simulink model "ts_b02f_log"  (R2024b)
settings: Solver=FixedStepDiscrete  StartTime=0.0  StopTime=10  FixedStep=Ts  RelTol=1e-4
PreLoadFcn:
  | Ts=50e-6;
undefined symbols (not defined in the file): D1, Delta, DiscIntNeverNeededParam
libraries: simulink x22, spsSecondOrderFilterLib x14, spsThreePhaseVIMeasurementLib x7, spsabctodq0Lib x6, spsThreePhaseSeriesRLCLoadLib x5, spsPowerPLLDrivenPositiveSequenceLib x4, spsStairGeneratorLib x4, spsThreePhaseTransformerTwoWindingsLib x3, spsDCVoltageSourceLib x3, spsThreePhaseSeriesRLCBranchLib x3, spsPWMGeneratorPulseAveragingLib x3, spsTwoLevelConverterLib x3
(part 1 of 3)
settings Model: Creator=The MathWorks, Inc.  LastModifiedBy=sande
settings SolverCC: AlgebraicLoopSolver=TrustRegion
settings DataIOCC: SaveOutput=off  DSMLogging=off  SaveTime=off  ReturnWorkspaceOutputs=off  SignalLoggingName=SignalLog
settings DebuggingCC: UnconnectedInputMsg=warning  UnconnectedOutputMsg=warning  UnconnectedLineMsg=warning  ArithmeticOperatorsInVariantConditions=warning
settings ModelReferenceCC: EnableRefExpFcnMdlSchedulingChecks=on
settings SFSimCC: CustomCodeUndefinedFunction=UseInterfaceOnly
settings RTWCC: GPUComputeCapability=3.5  DLArmComputeVersion=19.05

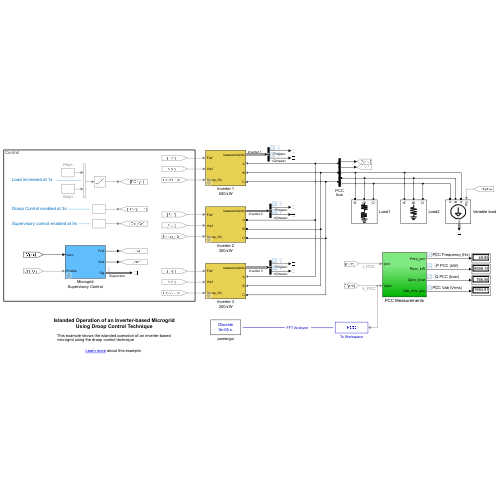
[thumbnail: Simulink's stored preview of the top-level diagram]
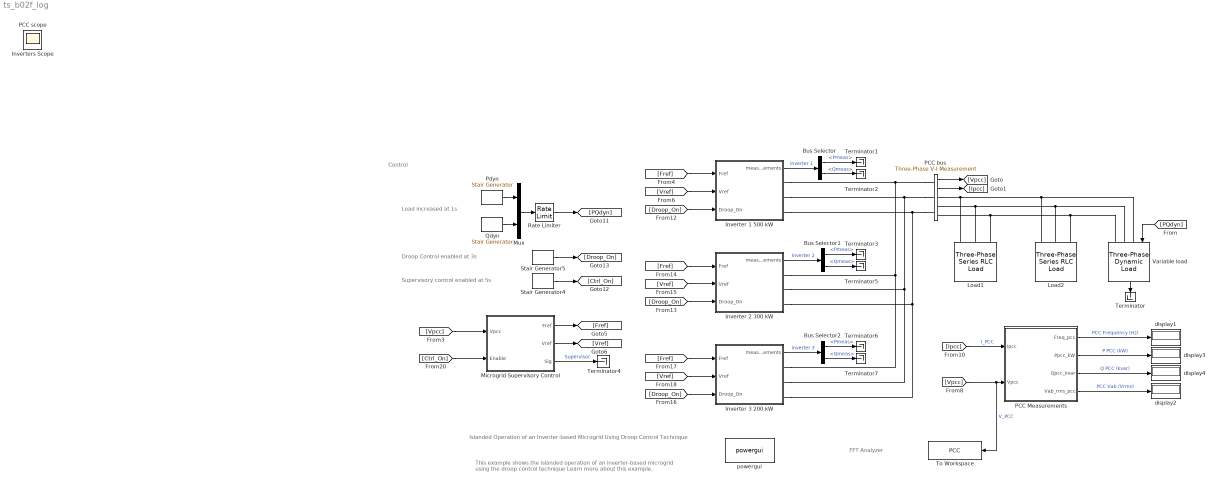
== system ts_b02f_log ==
  note: This example shows the islanded operation of an inverter-based microgrid using the droop control technique
      |
      | Learn more about this example.
  note: FFT Analyzer
  note: Control
  note: Islanded Operation of an Inverter-based Microgrid
      | Using Droop Control Technique
  note: Load increased at 1s
  note: Supervisory control enabled at 5s
  note: Droop Control enabled at 3s
  Bus Selector : BusSelector  OutputSignals=Control.Pmeas,Control.Qmeas
  Bus Selector1 : BusSelector  OutputSignals=Control.Pmeas,Control.Qmeas
  Bus Selector2 : BusSelector  OutputSignals=Control.Pmeas,Control.Qmeas
  Inverter 1 500 kW : Subsystem  mask(Grid-Forming Inverter with droop control){Pnom=5.874e+06, Fnom=50, Vnom_prim=22e3, Vnom_sec=480, Vnom_dc=1000, Frequency_Droop=1, Voltage_Droop=4, Kp_Vreg=2, Ki_Vreg=14, Kp_Ireg=0.3, Ki_Ireg=20, RLff=[ 0.004, 0.21], Fsw=2700, CarrierPhase=90, fn_Filter=500, Ts=Ts}
      mask prompts: Pnom "Power (VA)"; Fnom "Frequency (Hz)"; Vnom_prim "Primary line voltage (Vrms)"; Vnom_sec "Secondary line voltage (Vrms)"; Vnom_dc "DC link voltage (V)"; Frequency_Droop "Frequency droop (%)"; Voltage_Droop "Voltage droop (%)"; Kp_Vreg "Proportional gain"; Ki_Vreg "Integral gain"; Kp_Ireg "Proportional gain"; Ki_Ireg "Integral gain"; RLff "Feedforward coefficients (pu)"; Fsw "Switching frequency (Hz)"; CarrierPhase "Carrier initial phase (degrees)"; fn_Filter "Measurement filters fn (Hz)"; Ts "Sample time (s)"
      mask init:
      | Rff=RLff(1);
      | Lff=RLff(2);
      mask DialogControl Container4 Prompt: Nominal Values:
      mask DialogControl Container8 Prompt: Droop Values
      mask DialogControl Container7 Prompt: Voltage Regulators
      mask DialogControl Container10 Prompt: Current Regulators
      mask DialogControl Ts1 Prompt: PWM Generator
  Inverter 2 300 kW : Subsystem  mask(Grid-Forming Inverter with droop control){Pnom=5.874e+06, Fnom=50, Vnom_prim=22e3, Vnom_sec=480, Vnom_dc=1000, Frequency_Droop=1, Voltage_Droop=4, Kp_Vreg=2, Ki_Vreg=10, Kp_Ireg=0.3, Ki_Ireg=20, RLff=[ 0.004, 0.21], Fsw=2700, CarrierPhase=90, fn_Filter=500, Ts=Ts}
      mask prompts: Pnom "Power (VA)"; Fnom "Frequency (Hz)"; Vnom_prim "Primary line voltage (Vrms)"; Vnom_sec "Secondary line voltage (Vrms)"; Vnom_dc "DC link voltage (V)"; Frequency_Droop "Frequency droop (%)"; Voltage_Droop "Voltage droop (%)"; Kp_Vreg "Proportional gain"; Ki_Vreg "Integral gain"; Kp_Ireg "Proportional gain"; Ki_Ireg "Integral gain"; RLff "Feedforward coefficients (pu)"; Fsw "Switching frequency (Hz)"; CarrierPhase "Carrier initial phase (degrees)"; fn_Filter "Measurement filters fn (Hz)"; Ts "Sample time (s)"
      mask init:
      | Rff=RLff(1);
      | Lff=RLff(2);
      mask DialogControl Container4 Prompt: Nominal Values:
      mask DialogControl Container8 Prompt: Droop Values
      mask DialogControl Container7 Prompt: Voltage Regulators
      mask DialogControl Container10 Prompt: Current Regulators
      mask DialogControl Ts1 Prompt: PWM Generator
  Inverter 3 200 kW : Subsystem  mask(Grid-Forming Inverter with droop control){Pnom=5.874e+06, Fnom=50, Vnom_prim=22e3, Vnom_sec=480, Vnom_dc=1000, Frequency_Droop=1, Voltage_Droop=4, Kp_Vreg=2, Ki_Vreg=12, Kp_Ireg=0.3, Ki_Ireg=20, RLff=[ 0.004, 0.21], Fsw=2340, CarrierPhase=0, fn_Filter=500, Ts=Ts}
      mask prompts: Pnom "Power (VA)"; Fnom "Frequency (Hz)"; Vnom_prim "Primary line voltage (Vrms)"; Vnom_sec "Secondary line voltage (Vrms)"; Vnom_dc "DC link voltage (V)"; Frequency_Droop "Frequency droop (%)"; Voltage_Droop "Voltage droop (%)"; Kp_Vreg "Proportional gain"; Ki_Vreg "Integral gain"; Kp_Ireg "Proportional gain"; Ki_Ireg "Integral gain"; RLff "Feedforward coefficients (pu)"; Fsw "Switching frequency (Hz)"; CarrierPhase "Carrier initial phase (degrees)"; fn_Filter "Measurement filters fn (Hz)"; Ts "Sample time (s)"
      mask init:
      | Rff=RLff(1);
      | Lff=RLff(2);
      mask DialogControl Container4 Prompt: Nominal Values:
      mask DialogControl Container8 Prompt: Droop Values
      mask DialogControl Container7 Prompt: Voltage Regulators
      mask DialogControl Container10 Prompt: Current Regulators
      mask DialogControl Ts1 Prompt: PWM Generator
  Load1 : spsThreePhaseSeriesRLCLoadLib/Three-Phase Series RLC Load  LConnTagsString=A|B|C  Configuration=Y (grounded)  NominalVoltage=22e3  Vabc=[1e3 1e3 1e3]  Vabcp=[1e3 1e3 1e3]  NominalFrequency=50  UnbalancedPower=off  ActivePower=5e6  InductivePower=388172  CapacitivePower=0  Pabc=[10e3 9e3 11e3]  QLabc=[100 90 110]  QCabc=[100 90 110]  Pabcp=[10e3 9e3 11e3]  QLabcp=[100 90 110]  QCabcp=[100 90 110]  Measurements=None  LoadType=constant Z
  Load2 : spsThreePhaseSeriesRLCLoadLib/Three-Phase Series RLC Load  LConnTagsString=A|B|C  Configuration=Y (grounded)  NominalVoltage=22e3  Vabc=[1e3 1e3 1e3]  Vabcp=[1e3 1e3 1e3]  NominalFrequency=50  UnbalancedPower=off  ActivePower=0.05e6  InductivePower=0  CapacitivePower=0  Pabc=[10e3 9e3 11e3]  QLabc=[100 90 110]  QCabc=[100 90 110]  Pabcp=[10e3 9e3 11e3]  QLabcp=[100 90 110]  QCabcp=[100 90 110]  Measurements=None  LoadType=constant Z
  Microgrid Supervisory Control : Subsystem  mask(Microgrid Supervisory Control){Fnom=50, Vnom=22e3, Kp_Freg=0.03, Ki_Freg=2, Freg_Limits=[1.02, 0.98] * 50, Kp_Vreg=0.1, Ki_Vreg=7, Vreg_Limits=[1.04, 0.96] * 22e3, fn_Filter=10, Ts=Ts}
      mask prompts: Fnom "Frequency (Hz)"; Vnom "Line voltage (Vrms)"; Kp_Freg "Proportional gain"; Ki_Freg "Integral gain"; Freg_Limits "Output limits (Hz): [Upper Lower]"; Kp_Vreg "Proportional gain"; Ki_Vreg "Integral gain"; Vreg_Limits "Output limits (Hz): [Upper Lower]"; fn_Filter "Measurement filter fn (Hz)"; Ts "Sample time (s)"
      mask DialogControl Container4 Prompt: Nominal Values:
      mask DialogControl Container7 Prompt: Frequency Regulator
      mask DialogControl Container10 Prompt: Voltage Regulator
  Mux : Mux  Inputs=2
  PCC bus : spsThreePhaseVIMeasurementLib/Three-Phase V-I Measurement  VoltageMeasurement=phase-to-ground  SetLabelV=off  LabelV=Vabc  Vpu=off  VpuLL=off  CurrentMeasurement=yes  SetLabelI=off  LabelI=Iabc  Ipu=off  Pbase=100e6  Vbase=500e3  OutputType=Complex  PhasorSimulation=off  PSBequivalent=0
  PCC Measurements : Subsystem
  Pdyn : spsStairGeneratorLib/Stair Generator  t=[0, 1]  e=[0 4.95e6]  Ts=Ts
  Qdyn : spsStairGeneratorLib/Stair Generator  t=[0, 1]  e=[0 388172]  Ts=Ts
  Rate Limiter : RateLimiter  RisingSlewLimit=6.2e6  FallingSlewLimit=-6.2e6  SampleTimeMode=inherited
  Stair Generator4 : spsStairGeneratorLib/Stair Generator  t=[0, 5]  e=[0, 1]  Ts=Ts
  Stair Generator5 : spsStairGeneratorLib/Stair Generator  t=[0, 3]  e=[0, 1]  Ts=Ts
  Terminator{,1..7} (8 alike) : Terminator
  To Workspace : ToWorkspace  VariableName=PCC  SaveFormat=Structure With Time  SampleTime=-1
  Variable load : spsThreePhaseDynamicLoadLib/Three-Phase Dynamic Load  NominalVoltage=[ 22e3 50 ]  ActiveReactivePowers=[1e6 0]  PositiveSequence=[1 0]  ExternalControl=on  NpNq=[1.3 2]  TimeConstants="[0  0  0  0]"  MinimumVoltage=0.7  Tfilter=1e-4  LoadFlowParameters=[4,0,0,0,0]
      link override Model/PLL/Second-Order Filter: Vac_Init=[0, 0, 50]
  display{1..4} (4 alike) : Display
      settings: Format=bank  Decimation=500
  powergui : spspowerguiLib/powergui  Priority=2  SimulationMode=Discrete  SampleTime=Ts  frequency=50  Iterations=50  frequencyindice=0  Pbase=100e6  ErrMax=1e-4  UnitsV=kV  UnitsW=MW  buscounter=0  FunctionMessages=off  echomessages=off  EnableUseOfTLC=off  CurrentSourceSwitches=off  DisableSnubberDevices=off  DisableRonSwitches=off  DisableVfSwitches=off  DisplayEquations=off  AutomaticDiscreteSolvers=off  SolverType=Tustin/Backward Euler (TBE)  Interpol=off  ExternalGateDelay=off  methode=off  Ts=0  x0status=blocks  SPID=off  SwTol=0  HookPort=off  NonlinearTolerance=1e-4  nMaxIteration=100  ContinueOnMaxIteration=on  RestoreLinks=warning  ResistiveCurrentMeasurement=off  Frange=[0:2:500]  Ylog=off  Xlog=off  ShowGrid=off  save=off  variable=ZData  structure=ScopeData_VIpcc  ZoomFFT=on  StartTime=6.8  cycles=1  DisplayStyle=1  fundamental=50  FreqAxis=off  MaxFrequency=7000  frequencyindicesteady=1  RmsSteady=1  display=off
  Inverters Scope : Scope
  PCC scope : Scope
  wires:
  [Vref] -> Inverter 1 500 kW/2(Vref)
  [Fref] -> Inverter 1 500 kW/1(Fref)
  PCC bus/1 -> [Vpcc]
  PCC bus/2 -> [Ipcc]
  [Vpcc] -> Microgrid Supervisory Control/1(Vpcc)
  Microgrid Supervisory Control/1(Fref) -> [Fref]
  Microgrid Supervisory Control/2(Vref) -> [Vref]
  Microgrid Supervisory Control/3(Sig) -> Terminator4/1  "Supervisor"
  [Ipcc] -> PCC Measurements/1(Ipcc)  "I_PCC"
  [Vpcc] -> To Workspace/1, PCC Measurements/2(Vpcc)  "V_PCC"
  PCC Measurements/1(Freq_pcc) -> display1/1  "PCC Frequency (Hz)"
  PCC Measurements/4(Vab_rms_pcc) -> display2/1  "PCC Vab (Vrms)"
  [Droop_On] -> Inverter 1 500 kW/3(Droop_On)
  [Fref] -> Inverter 2 300 kW/1(Fref)
  [Vref] -> Inverter 2 300 kW/2(Vref)
  [Droop_On] -> Inverter 2 300 kW/3(Droop_On)
  [Fref] -> Inverter 3 200 kW/1(Fref)
  [Vref] -> Inverter 3 200 kW/2(Vref)
  [Droop_On] -> Inverter 3 200 kW/3(Droop_On)
  [Ctrl_On] -> Microgrid Supervisory Control/2(Enable)
  Variable load/1 -> Terminator/1
  [PQdyn] -> Variable load/1
  Mux/1 -> Rate Limiter/1
  Pdyn/1 -> Mux/1
  Qdyn/1 -> Mux/2
  Stair Generator5/1 -> [Droop_On]
  Stair Generator4/1 -> [Ctrl_On]
  Rate Limiter/1 -> [PQdyn]
  Inverter 1 500 kW/1(measurements) -> Bus Selector/1  "inverter 1"
  Inverter 2 300 kW/1(measurements) -> Bus Selector1/1  "inverter 2"
  Inverter 3 200 kW/1(measurements) -> Bus Selector2/1  "inverter 3"
  PCC Measurements/2(Ppcc_kW) -> display3/1  "P PCC (kW)"
  PCC Measurements/3(Qpcc_kvar) -> display4/1  "Q PCC (kvar)"
  Bus Selector/1 -> Terminator1/1  "<Pmeas>"
  Bus Selector/2 -> Terminator2/1  "<Qmeas>"
  Bus Selector1/1 -> Terminator3/1  "<Pmeas>"
  Bus Selector1/2 -> Terminator5/1  "<Qmeas>"
  Bus Selector2/1 -> Terminator6/1  "<Pmeas>"
  Bus Selector2/2 -> Terminator7/1  "<Qmeas>"
  connections:
  Load1/LConn1 -- Load2/LConn1 -- Variable load/LConn1 -- PCC bus/RConn1
  Load1/LConn2 -- Load2/LConn2 -- Variable load/LConn2 -- PCC bus/RConn2
  Load1/LConn3 -- Load2/LConn3 -- Variable load/LConn3 -- PCC bus/RConn3
  PCC bus/LConn2 -- Inverter 1 500 kW/RConn2 -- Inverter 2 300 kW/RConn2 -- Inverter 3 200 kW/RConn2
  PCC bus/LConn3 -- Inverter 1 500 kW/RConn3 -- Inverter 2 300 kW/RConn3 -- Inverter 3 200 kW/RConn3
  PCC bus/LConn1 -- Inverter 1 500 kW/RConn1 -- Inverter 2 300 kW/RConn1 -- Inverter 3 200 kW/RConn1

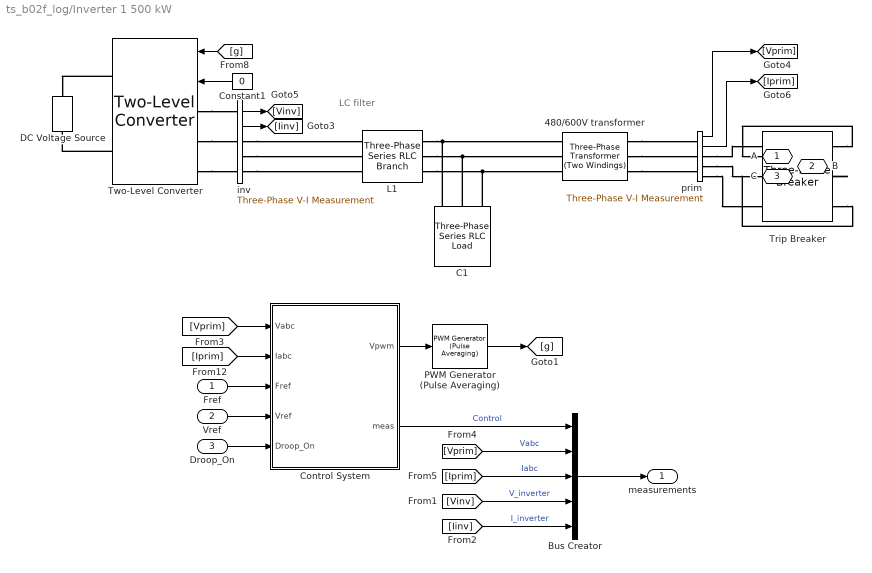
== system ts_b02f_log/Inverter 1 500 kW ==
  note: LC filter
  Fref : Inport  PortDimensions=1
  Vref : Inport  Port=2  PortDimensions=1
  Droop_On : Inport  Port=3  PortDimensions=1
  480/600V transformer : spsThreePhaseTransformerTwoWindingsLib/Three-Phase Transformer (Two Windings)  Winding1Connection=Yg  Winding2Connection=Delta (D1)  CoreType=Three single-phase transformers  SetSaturation=off  Hysteresis=off  DataFile='hysteresis'  SetInitialFlux=off  Measurements=None  UNITS=pu  NominalPower=[Pnom*1.1 , Fnom ]  Winding1=[ Vnom_prim , 0.0015 , 0.03]  Winding2=[Vnom_sec , 0.0015 , 0.03 ]  Rm=200  Lm=200  L0=0.5  Saturation=[ 0,0 ; 0.0024,1.2 ; 1.0,1.52 ]  InitialFluxes=[ 0.8 , -0.8 , 0.7 ]  BreakLoop=off  DiscreteSolver=Trapezoidal iterative  DataType=off  TransfoNumber=0
  Bus Creator : BusCreator  Inputs=5
  C1 : spsThreePhaseSeriesRLCLoadLib/Three-Phase Series RLC Load  LConnTagsString=A|B|C  Configuration=Y (grounded)  NominalVoltage=Vnom_sec  Vabc=[1e3 1e3 1e3]  Vabcp=[1e3 1e3 1e3]  NominalFrequency=Fnom  UnbalancedPower=off  ActivePower=0.05*Pnom/50  InductivePower=0  CapacitivePower=0.05*Pnom  Pabc=[10e3 9e3 11e3]  QLabc=[100 90 110]  QCabc=[100 90 110]  Pabcp=[10e3 9e3 11e3]  QLabcp=[100 90 110]  QCabcp=[100 90 110]  Measurements=None  LoadType=constant Z
  Constant1 : Constant  Value=0
  Control System : Subsystem  mask(Inverter Control){Pnom=Pnom, Fnom=Fnom, Vnom_prim=Vnom_prim, Vnom_sec=Vnom_sec, Vnom_dc=Vnom_dc, Frequency_Droop=Frequency_Droop, Voltage_Droop=Voltage_Droop, Kp_Vreg=Kp_Vreg, Ki_Vreg=Ki_Vreg, fn_Filter=fn_Filter, Kp_Ireg=Kp_Ireg, Ki_Ireg=Ki_Ireg, RLff=[ Rff Lff], Ts=Ts}
      mask prompts: Pnom "Power (VA)"; Fnom "Frequency (Hz)"; Vnom_prim "Primary voltage (Vrms)"; Vnom_sec "Secondary voltage (Vrms)"; Vnom_dc "DC voltage (V)"; Frequency_Droop "Frequency droop (%)"; Voltage_Droop "Voltage droop (%)"; Kp_Vreg "Proportional gain"; Ki_Vreg "Integral gain"; fn_Filter "Measurement filter fn (Hz)"; Kp_Ireg "Proportional gain"; Ki_Ireg "Integral gain"; RLff "Feedforward Values [Rff Lff] (pu)"; Ts "Control sample time:"
      mask init:
      | Rff=RLff(1);
      | Lff=RLff(2);
      | Limits_Ireg=[1.25, -1.25];
      | Limits_Vreg=[1.25, -1.25];
      mask DialogControl Container4 Prompt: Nominal Values:
      mask DialogControl Container8 Prompt: Droop Values
      mask DialogControl Container9 Prompt: Voltage regulators
      mask DialogControl Container6 Prompt: Current regulators:
      mask DialogControl Ts1 Prompt: Sample time (s)
  DC Voltage Source : spsDCVoltageSourceLib/DC Voltage Source  Amplitude=1000  Measurements=None
  L1 : spsThreePhaseSeriesRLCBranchLib/Three-Phase Series RLC Branch  LConnTagsString=A|B|C  RConnTagsString=A|B|C  BranchType=RL  Resistance=0.15 * (Vnom_sec^2/Pnom)/100  Inductance=0.15 * (Vnom_sec^2/Pnom/2/pi/Fnom)  Capacitance=inf  Measurements=None
  PWM Generator (Pulse Averaging) : spsPWMGeneratorPulseAveragingLib/PWM Generator (Pulse Averaging)  GeneratorType=Two-level, three-phase  Fc=Fsw  InitialPhase=CarrierPhase  Ts=Ts
  Trip Breaker : spsThreePhaseBreakerLib/Three-Phase Breaker  InitialState=closed  SwitchA=on  SwitchB=on  SwitchC=on  SwitchTimes=[6]  External=off  BreakerResistance=0.01  SnubberResistance=1e6  SnubberCapacitance=inf  Measurements=None
  Two-Level Converter : spsTwoLevelConverterLib/Two-Level Converter  ModelType=Switching function  Ron=1e-3  Rs=1e6  Cs=inf  Vforward=[0,0]  Ron_Diode=1e-3  Rs_Diode=1e6  Cs_Diode=inf  Vf_Diode=0  Rs_CurrentSource=inf  Ron_ACsource=1e-3
  inv : spsThreePhaseVIMeasurementLib/Three-Phase V-I Measurement  VoltageMeasurement=phase-to-ground  SetLabelV=off  LabelV=Vabc_B1  Vpu=off  VpuLL=off  CurrentMeasurement=yes  SetLabelI=off  LabelI=Iabc_B1  Ipu=off  Pbase=100e6  Vbase=500e3  OutputType=Magnitude  PhasorSimulation=off  PSBequivalent=0
  prim : spsThreePhaseVIMeasurementLib/Three-Phase V-I Measurement  VoltageMeasurement=phase-to-ground  SetLabelV=off  LabelV=Vabc_B1  Vpu=off  VpuLL=off  CurrentMeasurement=yes  SetLabelI=off  LabelI=Iabc_B1  Ipu=off  Pbase=100e6  Vbase=500e3  OutputType=Magnitude  PhasorSimulation=off  PSBequivalent=0
  A : PMIOPort  Side=Right
  B : PMIOPort  Port=2  Side=Right
  C : PMIOPort  Port=3  Side=Right
  measurements : Outport
  wires:
  Bus Creator/1 -> measurements/1
  [Iinv] -> Bus Creator/5  "I_inverter"
  [Vinv] -> Bus Creator/4  "V_inverter"
  [Iprim] -> Bus Creator/3  "Iabc"
  [Vprim] -> Bus Creator/2  "Vabc"
  Control System/1(Vpwm) -> PWM Generator (Pulse Averaging)/1
  inv/2 -> [Iinv]
  PWM Generator (Pulse Averaging)/1 -> [g]
  inv/1 -> [Vinv]
  [g] -> Two-Level Converter/1
  Constant1/1 -> Two-Level Converter/2
  Fref/1 -> Control System/3(Fref)
  Vref/1 -> Control System/4(Vref)
  Control System/2(meas) -> Bus Creator/1  "Control"
  Droop_On/1 -> Control System/5(Droop_On)
  prim/2 -> [Iprim]
  prim/1 -> [Vprim]
  [Vprim] -> Control System/1(Vabc)
  [Iprim] -> Control System/2(Iabc)
  connections:
  L1/RConn2 -- 480/600V transformer/RConn2 -- C1/LConn2
  L1/RConn1 -- 480/600V transformer/RConn1 -- C1/LConn1
  L1/RConn3 -- 480/600V transformer/RConn3 -- C1/LConn3
  Two-Level Converter/RConn1 -- DC Voltage Source/RConn1
  inv/RConn3 -- L1/LConn3
  Two-Level Converter/LConn3 -- inv/LConn3
  inv/RConn1 -- L1/LConn1
  Two-Level Converter/LConn2 -- inv/LConn2
  inv/RConn2 -- L1/LConn2
  Two-Level Converter/LConn1 -- inv/LConn1
  Two-Level Converter/RConn2 -- DC Voltage Source/LConn1
  480/600V transformer/LConn2 -- prim/LConn2
  480/600V transformer/LConn1 -- prim/LConn1
  480/600V transformer/LConn3 -- prim/LConn3
  prim/RConn1 -- Trip Breaker/LConn1
  Trip Breaker/RConn1 -- A/RConn1
  prim/RConn2 -- Trip Breaker/LConn2
  Trip Breaker/RConn2 -- B/RConn1
  prim/RConn3 -- Trip Breaker/LConn3
  Trip Breaker/RConn3 -- C/RConn1

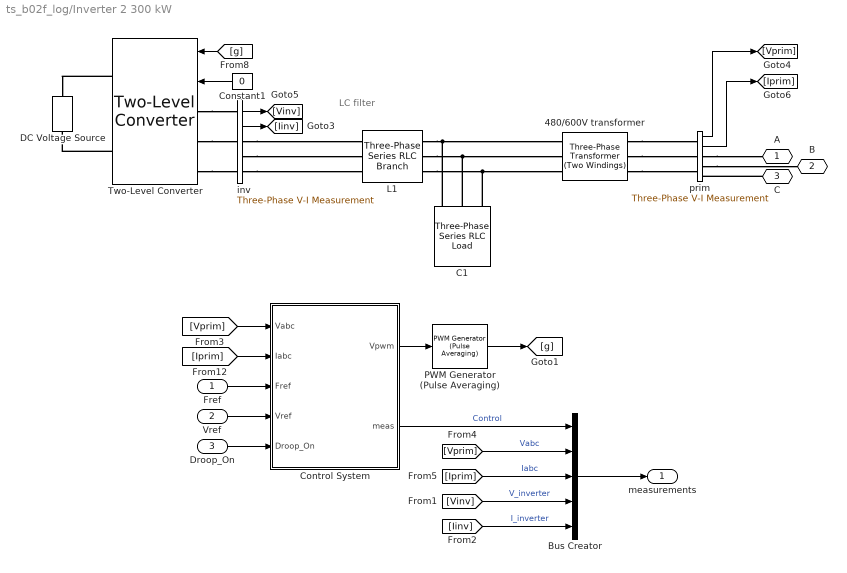
== system ts_b02f_log/Inverter 2 300 kW ==
  note: LC filter
  Fref : Inport  PortDimensions=1
  Vref : Inport  Port=2  PortDimensions=1
  Droop_On : Inport  Port=3  PortDimensions=1
  480/600V transformer : spsThreePhaseTransformerTwoWindingsLib/Three-Phase Transformer (Two Windings)  Winding1Connection=Yg  Winding2Connection=Delta (D1)  CoreType=Three single-phase transformers  SetSaturation=off  Hysteresis=off  DataFile='hysteresis'  SetInitialFlux=off  Measurements=None  UNITS=pu  NominalPower=[Pnom*1.1 , Fnom ]  Winding1=[ Vnom_prim , 0.0015 , 0.03]  Winding2=[Vnom_sec , 0.0015 , 0.03 ]  Rm=200  Lm=200  L0=0.5  Saturation=[ 0,0 ; 0.0024,1.2 ; 1.0,1.52 ]  InitialFluxes=[ 0.8 , -0.8 , 0.7 ]  BreakLoop=off  DiscreteSolver=Trapezoidal iterative  DataType=off  TransfoNumber=0
  Bus Creator : BusCreator  Inputs=5
  C1 : spsThreePhaseSeriesRLCLoadLib/Three-Phase Series RLC Load  LConnTagsString=A|B|C  Configuration=Y (grounded)  NominalVoltage=Vnom_sec  Vabc=[1e3 1e3 1e3]  Vabcp=[1e3 1e3 1e3]  NominalFrequency=Fnom  UnbalancedPower=off  ActivePower=0.05*Pnom/50  InductivePower=0  CapacitivePower=0.05*Pnom  Pabc=[10e3 9e3 11e3]  QLabc=[100 90 110]  QCabc=[100 90 110]  Pabcp=[10e3 9e3 11e3]  QLabcp=[100 90 110]  QCabcp=[100 90 110]  Measurements=None  LoadType=constant Z
  Constant1 : Constant  Value=0
  Control System : Subsystem  mask(Inverter Control){Pnom=Pnom, Fnom=Fnom, Vnom_prim=Vnom_prim, Vnom_sec=Vnom_sec, Vnom_dc=Vnom_dc, Frequency_Droop=Frequency_Droop, Voltage_Droop=Voltage_Droop, Kp_Vreg=Kp_Vreg, Ki_Vreg=Ki_Vreg, fn_Filter=fn_Filter, Kp_Ireg=Kp_Ireg, Ki_Ireg=Ki_Ireg, RLff=[ Rff Lff], Ts=Ts}
      mask prompts: Pnom "Power (VA)"; Fnom "Frequency (Hz)"; Vnom_prim "Primary voltage (Vrms)"; Vnom_sec "Secondary voltage (Vrms)"; Vnom_dc "DC voltage (V)"; Frequency_Droop "Frequency droop (%)"; Voltage_Droop "Voltage droop (%)"; Kp_Vreg "Proportional gain"; Ki_Vreg "Integral gain"; fn_Filter "Measurement filter fn (Hz)"; Kp_Ireg "Proportional gain"; Ki_Ireg "Integral gain"; RLff "Feedforward Values [Rff Lff] (pu)"; Ts "Control sample time:"
      mask init:
      | Rff=RLff(1);
      | Lff=RLff(2);
      | Limits_Ireg=[1.25, -1.25];
      | Limits_Vreg=[1.25, -1.25];
      mask DialogControl Container4 Prompt: Nominal Values:
      mask DialogControl Container8 Prompt: Droop Values
      mask DialogControl Container9 Prompt: Voltage regulators
      mask DialogControl Container6 Prompt: Current regulators:
      mask DialogControl Ts1 Prompt: Sample time (s)
  DC Voltage Source : spsDCVoltageSourceLib/DC Voltage Source  Amplitude=1000  Measurements=None
  L1 : spsThreePhaseSeriesRLCBranchLib/Three-Phase Series RLC Branch  LConnTagsString=A|B|C  RConnTagsString=A|B|C  BranchType=RL  Resistance=0.15 * (Vnom_sec^2/Pnom)/100  Inductance=0.15 * (Vnom_sec^2/Pnom/2/pi/Fnom)  Capacitance=inf  Measurements=None
  PWM Generator (Pulse Averaging) : spsPWMGeneratorPulseAveragingLib/PWM Generator (Pulse Averaging)  GeneratorType=Two-level, three-phase  Fc=Fsw  InitialPhase=CarrierPhase  Ts=Ts
  Two-Level Converter : spsTwoLevelConverterLib/Two-Level Converter  ModelType=Switching function  Ron=1e-3  Rs=1e6  Cs=inf  Vforward=[0,0]  Ron_Diode=1e-3  Rs_Diode=1e6  Cs_Diode=inf  Vf_Diode=0  Rs_CurrentSource=inf  Ron_ACsource=1e-3
  inv : spsThreePhaseVIMeasurementLib/Three-Phase V-I Measurement  VoltageMeasurement=phase-to-ground  SetLabelV=off  LabelV=Vabc_B1  Vpu=off  VpuLL=off  CurrentMeasurement=yes  SetLabelI=off  LabelI=Iabc_B1  Ipu=off  Pbase=100e6  Vbase=500e3  OutputType=Magnitude  PhasorSimulation=off  PSBequivalent=0
  prim : spsThreePhaseVIMeasurementLib/Three-Phase V-I Measurement  VoltageMeasurement=phase-to-ground  SetLabelV=off  LabelV=Vabc_B1  Vpu=off  VpuLL=off  CurrentMeasurement=yes  SetLabelI=off  LabelI=Iabc_B1  Ipu=off  Pbase=100e6  Vbase=500e3  OutputType=Magnitude  PhasorSimulation=off  PSBequivalent=0
  A : PMIOPort  Side=Right
  B : PMIOPort  Port=2  Side=Right
  C : PMIOPort  Port=3  Side=Right
  measurements : Outport
  wires:
  Bus Creator/1 -> measurements/1
  [Iinv] -> Bus Creator/5  "I_inverter"
  [Vinv] -> Bus Creator/4  "V_inverter"
  [Iprim] -> Bus Creator/3  "Iabc"
  [Vprim] -> Bus Creator/2  "Vabc"
  Control System/1(Vpwm) -> PWM Generator (Pulse Averaging)/1
  inv/2 -> [Iinv]
  PWM Generator (Pulse Averaging)/1 -> [g]
  inv/1 -> [Vinv]
  [g] -> Two-Level Converter/1
  Constant1/1 -> Two-Level Converter/2
  Fref/1 -> Control System/3(Fref)
  Vref/1 -> Control System/4(Vref)
  Control System/2(meas) -> Bus Creator/1  "Control"
  Droop_On/1 -> Control System/5(Droop_On)
  prim/2 -> [Iprim]
  prim/1 -> [Vprim]
  [Vprim] -> Control System/1(Vabc)
  [Iprim] -> Control System/2(Iabc)
  connections:
  L1/RConn2 -- 480/600V transformer/RConn2 -- C1/LConn2
  L1/RConn1 -- 480/600V transformer/RConn1 -- C1/LConn1
  L1/RConn3 -- 480/600V transformer/RConn3 -- C1/LConn3
  Two-Level Converter/RConn1 -- DC Voltage Source/RConn1
  inv/RConn3 -- L1/LConn3
  Two-Level Converter/LConn3 -- inv/LConn3
  inv/RConn1 -- L1/LConn1
  Two-Level Converter/LConn2 -- inv/LConn2
  inv/RConn2 -- L1/LConn2
  Two-Level Converter/LConn1 -- inv/LConn1
  prim/RConn1 -- A/RConn1
  prim/RConn2 -- B/RConn1
  C/RConn1 -- prim/RConn3
  Two-Level Converter/RConn2 -- DC Voltage Source/LConn1
  480/600V transformer/LConn2 -- prim/LConn2
  480/600V transformer/LConn1 -- prim/LConn1
  480/600V transformer/LConn3 -- prim/LConn3

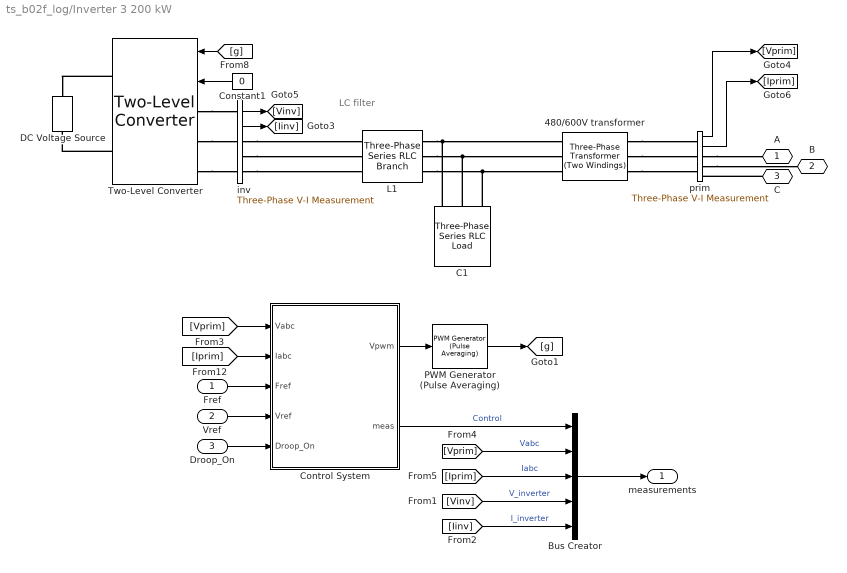
== system ts_b02f_log/Inverter 3 200 kW ==
  note: LC filter
  Fref : Inport  PortDimensions=1
  Vref : Inport  Port=2  PortDimensions=1
  Droop_On : Inport  Port=3  PortDimensions=1
  480/600V transformer : spsThreePhaseTransformerTwoWindingsLib/Three-Phase Transformer (Two Windings)  Winding1Connection=Yg  Winding2Connection=Delta (D1)  CoreType=Three single-phase transformers  SetSaturation=off  Hysteresis=off  DataFile='hysteresis'  SetInitialFlux=off  Measurements=None  UNITS=pu  NominalPower=[Pnom*1.1 , Fnom ]  Winding1=[ Vnom_prim , 0.0015 , 0.03]  Winding2=[Vnom_sec , 0.0015 , 0.03 ]  Rm=200  Lm=200  L0=0.5  Saturation=[ 0,0 ; 0.0024,1.2 ; 1.0,1.52 ]  InitialFluxes=[ 0.8 , -0.8 , 0.7 ]  BreakLoop=off  DiscreteSolver=Trapezoidal iterative  DataType=off  TransfoNumber=0
  Bus Creator : BusCreator  Inputs=5
  C1 : spsThreePhaseSeriesRLCLoadLib/Three-Phase Series RLC Load  LConnTagsString=A|B|C  Configuration=Y (grounded)  NominalVoltage=Vnom_sec  Vabc=[1e3 1e3 1e3]  Vabcp=[1e3 1e3 1e3]  NominalFrequency=Fnom  UnbalancedPower=off  ActivePower=0.05*Pnom/50  InductivePower=0  CapacitivePower=0.05*Pnom  Pabc=[10e3 9e3 11e3]  QLabc=[100 90 110]  QCabc=[100 90 110]  Pabcp=[10e3 9e3 11e3]  QLabcp=[100 90 110]  QCabcp=[100 90 110]  Measurements=None  LoadType=constant Z
  Constant1 : Constant  Value=0
  Control System : Subsystem  mask(Inverter Control){Pnom=Pnom, Fnom=Fnom, Vnom_prim=Vnom_prim, Vnom_sec=Vnom_sec, Vnom_dc=Vnom_dc, Frequency_Droop=Frequency_Droop, Voltage_Droop=Voltage_Droop, Kp_Vreg=Kp_Vreg, Ki_Vreg=Ki_Vreg, fn_Filter=fn_Filter, Kp_Ireg=Kp_Ireg, Ki_Ireg=Ki_Ireg, RLff=[ Rff Lff], Ts=Ts}
      mask prompts: Pnom "Power (VA)"; Fnom "Frequency (Hz)"; Vnom_prim "Primary voltage (Vrms)"; Vnom_sec "Secondary voltage (Vrms)"; Vnom_dc "DC voltage (V)"; Frequency_Droop "Frequency droop (%)"; Voltage_Droop "Voltage droop (%)"; Kp_Vreg "Proportional gain"; Ki_Vreg "Integral gain"; fn_Filter "Measurement filter fn (Hz)"; Kp_Ireg "Proportional gain"; Ki_Ireg "Integral gain"; RLff "Feedforward Values [Rff Lff] (pu)"; Ts "Control sample time:"
      mask init:
      | Rff=RLff(1);
      | Lff=RLff(2);
      | Limits_Ireg=[1.25, -1.25];
      | Limits_Vreg=[1.25, -1.25];
      mask DialogControl Container4 Prompt: Nominal Values:
      mask DialogControl Container8 Prompt: Droop Values
      mask DialogControl Container9 Prompt: Voltage regulators
      mask DialogControl Container6 Prompt: Current regulators:
      mask DialogControl Ts1 Prompt: Sample time (s)
  DC Voltage Source : spsDCVoltageSourceLib/DC Voltage Source  Amplitude=1000  Measurements=None
  L1 : spsThreePhaseSeriesRLCBranchLib/Three-Phase Series RLC Branch  LConnTagsString=A|B|C  RConnTagsString=A|B|C  BranchType=RL  Resistance=0.15 * (Vnom_sec^2/Pnom)/100  Inductance=0.15 * (Vnom_sec^2/Pnom/2/pi/Fnom)  Capacitance=inf  Measurements=None
  PWM Generator (Pulse Averaging) : spsPWMGeneratorPulseAveragingLib/PWM Generator (Pulse Averaging)  GeneratorType=Two-level, three-phase  Fc=Fsw  InitialPhase=CarrierPhase  Ts=Ts
  Two-Level Converter : spsTwoLevelConverterLib/Two-Level Converter  ModelType=Switching function  Ron=1e-3  Rs=1e6  Cs=inf  Vforward=[0,0]  Ron_Diode=1e-3  Rs_Diode=1e6  Cs_Diode=inf  Vf_Diode=0  Rs_CurrentSource=inf  Ron_ACsource=1e-3
  inv : spsThreePhaseVIMeasurementLib/Three-Phase V-I Measurement  VoltageMeasurement=phase-to-ground  SetLabelV=off  LabelV=Vabc_B1  Vpu=off  VpuLL=off  CurrentMeasurement=yes  SetLabelI=off  LabelI=Iabc_B1  Ipu=off  Pbase=100e6  Vbase=500e3  OutputType=Magnitude  PhasorSimulation=off  PSBequivalent=0
  prim : spsThreePhaseVIMeasurementLib/Three-Phase V-I Measurement  VoltageMeasurement=phase-to-ground  SetLabelV=off  LabelV=Vabc_B1  Vpu=off  VpuLL=off  CurrentMeasurement=yes  SetLabelI=off  LabelI=Iabc_B1  Ipu=off  Pbase=100e6  Vbase=500e3  OutputType=Magnitude  PhasorSimulation=off  PSBequivalent=0
  A : PMIOPort  Side=Right
  B : PMIOPort  Port=2  Side=Right
  C : PMIOPort  Port=3  Side=Right
  measurements : Outport
  wires:
  Bus Creator/1 -> measurements/1
  [Iinv] -> Bus Creator/5  "I_inverter"
  [Vinv] -> Bus Creator/4  "V_inverter"
  [Iprim] -> Bus Creator/3  "Iabc"
  [Vprim] -> Bus Creator/2  "Vabc"
  Control System/1(Vpwm) -> PWM Generator (Pulse Averaging)/1
  inv/2 -> [Iinv]
  PWM Generator (Pulse Averaging)/1 -> [g]
  inv/1 -> [Vinv]
  [g] -> Two-Level Converter/1
  Constant1/1 -> Two-Level Converter/2
  Fref/1 -> Control System/3(Fref)
  Vref/1 -> Control System/4(Vref)
  Control System/2(meas) -> Bus Creator/1  "Control"
  Droop_On/1 -> Control System/5(Droop_On)
  prim/2 -> [Iprim]
  prim/1 -> [Vprim]
  [Vprim] -> Control System/1(Vabc)
  [Iprim] -> Control System/2(Iabc)
  connections:
  L1/RConn2 -- 480/600V transformer/RConn2 -- C1/LConn2
  L1/RConn1 -- 480/600V transformer/RConn1 -- C1/LConn1
  L1/RConn3 -- 480/600V transformer/RConn3 -- C1/LConn3
  Two-Level Converter/RConn1 -- DC Voltage Source/RConn1
  inv/RConn3 -- L1/LConn3
  Two-Level Converter/LConn3 -- inv/LConn3
  inv/RConn1 -- L1/LConn1
  Two-Level Converter/LConn2 -- inv/LConn2
  inv/RConn2 -- L1/LConn2
  Two-Level Converter/LConn1 -- inv/LConn1
  prim/RConn1 -- A/RConn1
  prim/RConn2 -- B/RConn1
  C/RConn1 -- prim/RConn3
  Two-Level Converter/RConn2 -- DC Voltage Source/LConn1
  480/600V transformer/LConn2 -- prim/LConn2
  480/600V transformer/LConn1 -- prim/LConn1
  480/600V transformer/LConn3 -- prim/LConn3

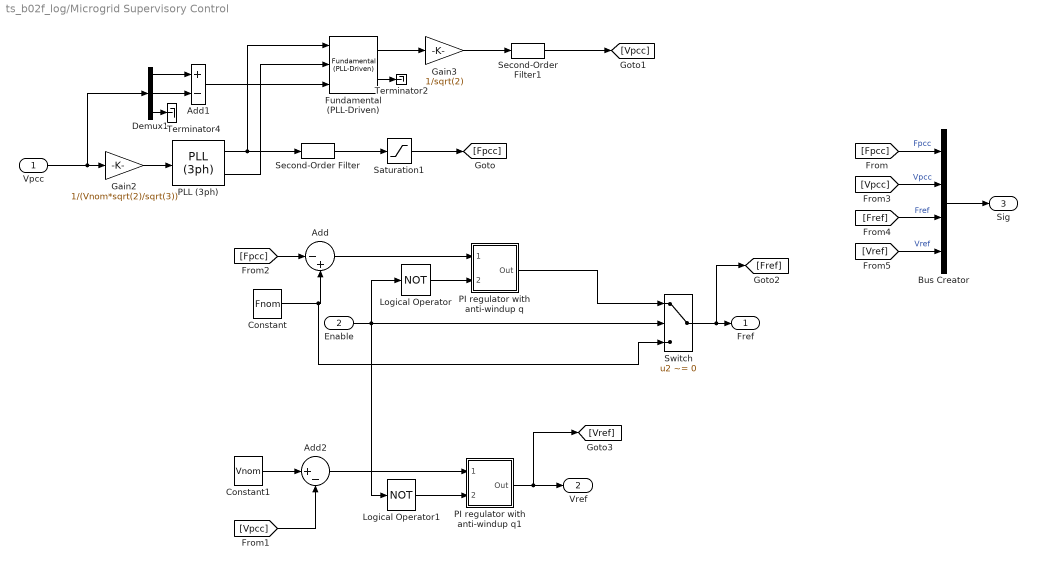
== system ts_b02f_log/Microgrid Supervisory Control ==
  Vpcc : Inport
  Enable : Inport  Port=2
  Add : Sum  Inputs=|-+
  Add1 : Sum  Inputs=+-
  Add2 : Sum  Inputs=|+-
  Bus Creator : BusCreator  Inputs=4
  Constant : Constant  Value=Fnom  SampleTime=Ts
  Constant1 : Constant  Value=Vnom  SampleTime=Ts
  Demux1 : Demux  Outputs=3
  Fundamental (PLL-Driven) : spsFundamentalPLLDrivenLib/Fundamental (PLL-Driven)  Finit=Fnom  Fmin=45  InInit=[1, 0]  Ts=Ts
  Gain2 : Gain  Gain=1/(Vnom*sqrt(2)/sqrt(3))
  Gain3 : Gain  Gain=1/sqrt(2)
  Logical Operator : Logic  Operator=NOT  AllPortsSameDT=off  OutDataTypeStr=boolean
  Logical Operator1 : Logic  Operator=NOT  AllPortsSameDT=off  OutDataTypeStr=boolean
  PI regulator with anti-windup q : Subsystem  DialogController=POWERSYS.PowerSysDialog  mask(Discrete PI Controller){Kp=Kp_Freg, Ki=Ki_Freg, Par_Limits=Freg_Limits, Init=Fnom, Ts=Ts}
      mask prompts: Kp "Proportional gain (Kp):"; Ki "Integral gain (Ki):"; Par_Limits "Output limits: [ Upper   Lower ]"; Init "Output initial value:"; Ts "Sample time:"
      mask help: This block implements a discrete PI controller.
      mask init:
      | UpperLimit=Par_Limits(1);
      | LowerLimit=Par_Limits(2);
      | power_initmask();
      mask Help: This block is part of a subset of blocks in the Extras library that does not have documentation associated with it, other than the block mask description.
      mask Display: disp('PI');
  PI regulator with anti-windup q1 : Subsystem  DialogController=POWERSYS.PowerSysDialog  mask(Discrete PI Controller){Kp=Kp_Vreg, Ki=Ki_Vreg, Par_Limits=Vreg_Limits, Init=Vnom, Ts=Ts}
      mask prompts: Kp "Proportional gain (Kp):"; Ki "Integral gain (Ki):"; Par_Limits "Output limits: [ Upper   Lower ]"; Init "Output initial value:"; Ts "Sample time:"
      mask help: This block implements a discrete PI controller.
      mask init:
      | UpperLimit=Par_Limits(1);
      | LowerLimit=Par_Limits(2);
      | power_initmask();
      mask Help: This block is part of a subset of blocks in the Extras library that does not have documentation associated with it, other than the block mask description.
      mask Display: disp('PI');
  PLL (3ph) : spsPLL3phLib/PLL (3ph)  Fmin=45  Par_Init=[0, Fnom]  ParK=[180, 3200, 1]  TcD=1e-4  MaxRateChangeFreq=12  FilterCutOffFreq=25  Ts=Ts  AGC=on
      link override Model/Second-Order Filter: Vac_Init=[0, 0, 50]
  Saturation1 : Saturate  UpperLimit=1.1*Fnom  LowerLimit=0.9*Fnom
  Second-Order Filter : spsSecondOrderFilterLib/Second-Order Filter  FilterType=Lowpass  Fo=fn_Filter  Zeta=1  Ts=Ts  Initialize=on  Vac_Init=[0, 0, 50]  Vdc_Init=Fnom  PlotResponse=off  FreqRange=[0, 500, 1]
  Second-Order Filter1 : spsSecondOrderFilterLib/Second-Order Filter  FilterType=Lowpass  Fo=fn_Filter  Zeta=1  Ts=Ts  Initialize=on  Vac_Init=[0, 0, 50]  Vdc_Init=Vnom  PlotResponse=off  FreqRange=[0, 500, 1]
  Switch : Switch  Criteria=u2 ~= 0  SaturateOnIntegerOverflow=off  InputSameDT=off
  Terminator2 : Terminator
  Terminator4 : Terminator
  Fref : Outport
  Vref : Outport  Port=2
  Sig : Outport  Port=3
  wires:
  [Vpcc] -> Add2/2
  Switch/1 -> [Fref], Fref/1
  Add2/1 -> PI regulator with anti-windup q1/1(Error)
  Second-Order Filter1/1 -> [Vpcc]
  [Fpcc] -> Add/1
  Second-Order Filter/1 -> Saturation1/1
  Saturation1/1 -> [Fpcc]
  Gain3/1 -> Second-Order Filter1/1
  PLL (3ph)/1 -> Fundamental (PLL-Driven)/1, Second-Order Filter/1
  [Vref] -> Bus Creator/4  "Vref"
  [Fpcc] -> Bus Creator/1  "Fpcc"
  [Fref] -> Bus Creator/3  "Fref"
  Demux1/2 -> Add1/2
  Constant/1 -> Switch/3, Add/2
  Demux1/1 -> Add1/1
  PI regulator with anti-windup q/1(Out) -> Switch/1
  Bus Creator/1 -> Sig/1
  PLL (3ph)/2 -> Fundamental (PLL-Driven)/2
  Gain2/1 -> PLL (3ph)/1
  Vpcc/1 -> Gain2/1, Demux1/1
  Fundamental (PLL-Driven)/2 -> Terminator2/1
  [Vpcc] -> Bus Creator/2  "Vpcc"
  Add/1 -> PI regulator with anti-windup q/1(Error)
  Enable/1 -> Logical Operator1/1, Logical Operator/1, Switch/2
  Logical Operator/1 -> PI regulator with anti-windup q/2(Reset)
  Constant1/1 -> Add2/1
  Fundamental (PLL-Driven)/1 -> Gain3/1
  PI regulator with anti-windup q1/1(Out) -> [Vref], Vref/1
  Demux1/3 -> Terminator4/1
  Logical Operator1/1 -> PI regulator with anti-windup q1/2(Reset)
  Add1/1 -> Fundamental (PLL-Driven)/3

== system ts_b02f_log/PCC Measurements ==
  Ipcc : Inport
  Vpcc : Inport  Port=2
  Add1 : Sum  Inputs=+-
  Demux1 : Demux  Outputs=3
  Fundamental (PLL-Driven) : spsFundamentalPLLDrivenLib/Fundamental (PLL-Driven)  Finit=50  Fmin=45  InInit=[22e3*sqrt(2), 0]  Ts=Ts
  Gain : Gain  Gain=1e-3
  Gain1 : Gain  Gain=1e-3
  Gain2 : Gain  Gain=1/(22e3*sqrt(2)/sqrt(3))
  Gain3 : Gain  Gain=1/sqrt(2)
  PLL (3ph) : spsPLL3phLib/PLL (3ph)  Fmin=45  Par_Init=[0, 50]  ParK=[180, 3200, 1]  TcD=1e-4  MaxRateChangeFreq=12  FilterCutOffFreq=25  Ts=Ts  AGC=on
      link override Model/Second-Order Filter: Vac_Init=[0, 0, 50]
  "Power (PLL-Driven, Positive-Sequence)" : spsPowerPLLDrivenPositiveSequenceLib/Power (PLL-Driven, Positive-Sequence)  Finit=50  Fmin=45  Vinit=[1, 0]  Iinit=[1, 0]  Ts=Ts
  Saturation1 : Saturate  UpperLimit=55  LowerLimit=45
  Terminator2 : Terminator
  Terminator4 : Terminator
  Freq_pcc : Outport
  Ppcc_kW : Outport  Port=2
  Qpcc_kvar : Outport  Port=3
  Vab_rms_pcc : Outport  Port=4
  wires:
  Ipcc/1 -> "Power (PLL-Driven, Positive-Sequence)"/4
  Demux1/2 -> Add1/2
  PLL (3ph)/2 -> Fundamental (PLL-Driven)/2, "Power (PLL-Driven, Positive-Sequence)"/2
  PLL (3ph)/1 -> Saturation1/1
  Demux1/3 -> Terminator4/1
  Demux1/1 -> Add1/1
  Fundamental (PLL-Driven)/2 -> Terminator2/1
  Gain2/1 -> PLL (3ph)/1
  "Power (PLL-Driven, Positive-Sequence)"/1 -> Gain/1
  Vpcc/1 -> Demux1/1, "Power (PLL-Driven, Positive-Sequence)"/3, Gain2/1
  Fundamental (PLL-Driven)/1 -> Gain3/1
  "Power (PLL-Driven, Positive-Sequence)"/2 -> Gain1/1
  Add1/1 -> Fundamental (PLL-Driven)/3
  Gain3/1 -> Vab_rms_pcc/1
  Gain/1 -> Ppcc_kW/1
  Gain1/1 -> Qpcc_kvar/1
  Saturation1/1 -> Freq_pcc/1, Fundamental (PLL-Driven)/1, "Power (PLL-Driven, Positive-Sequence)"/1

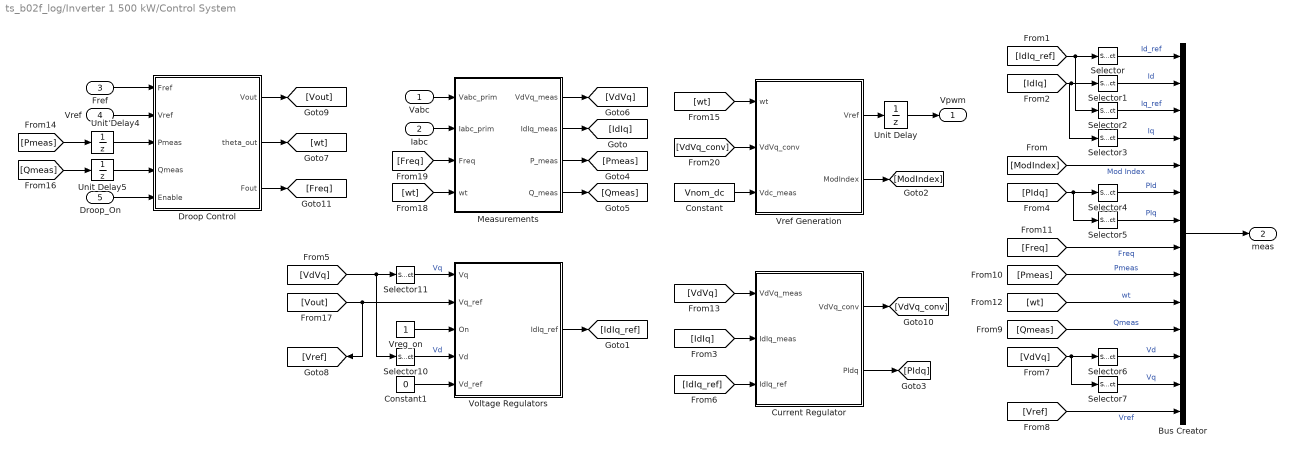
== system ts_b02f_log/Inverter 1 500 kW/Control System ==
  Vabc : Inport  PortDimensions=3
  Iabc : Inport  Port=2  PortDimensions=3
  Fref : Inport  Port=3  PortDimensions=1
  Vref : Inport  Port=4  PortDimensions=1
  Droop_On : Inport  Port=5
  Bus Creator : BusCreator  Inputs=14
  Constant : Constant  Value=Vnom_dc  SampleTime=Ts
  Constant1 : Constant  Value=0  SampleTime=Ts
  Current Regulator : Subsystem
  Droop Control : Subsystem
  Measurements : Subsystem
  Selector{,1,4,6,10} (5 alike) : Selector  InputPortWidth=2  IndexOptions=Index vector (dialog)  Indices=1  OutputSizes=1
  Selector{2..3,5,7,11} (5 alike) : Selector  InputPortWidth=2  IndexOptions=Index vector (dialog)  Indices=2  OutputSizes=1
  Unit Delay : UnitDelay  SampleTime=-1  HasFrameUpgradeWarning=on
  Unit Delay4 : UnitDelay  SampleTime=-1  HasFrameUpgradeWarning=on
  Unit Delay5 : UnitDelay  SampleTime=-1  HasFrameUpgradeWarning=on
  Voltage Regulators : Subsystem
  Vref Generation : Subsystem
  Vreg_on : Constant
  Vpwm : Outport  VectorParamsAs1DForOutWhenUnconnected=off
  meas : Outport  Port=2  VectorParamsAs1DForOutWhenUnconnected=off
  wires:
  Selector1/1 -> Bus Creator/2  "Id"
  Selector5/1 -> Bus Creator/7  "PIq"
  Selector4/1 -> Bus Creator/6  "PId"
  Vref Generation/1(Vref) -> Unit Delay/1
  Iabc/1 -> Measurements/2(Iabc_prim)
  Vref Generation/2(ModIndex) -> [ModIndex]
  Vreg_on/1 -> Voltage Regulators/3(On)
  [IdIq] -> Selector1/1, Selector3/1
  [Qmeas] -> Bus Creator/11  "Qmeas"
  Selector/1 -> Bus Creator/1  "Id_ref"
  [Freq] -> Bus Creator/8  "Freq"
  [wt] -> Bus Creator/10  "wt"
  Selector2/1 -> Bus Creator/3  "Iq_ref"
  Measurements/4(Q_meas) -> [Qmeas]
  [IdIq_ref] -> Current Regulator/3(IdIq_ref)
  [PIdq] -> Selector5/1, Selector4/1
  [Pmeas] -> Bus Creator/9  "Pmeas"
  Vabc/1 -> Measurements/1(Vabc_prim)
  Current Regulator/2(PIdq) -> [PIdq]
  [Vout] -> Voltage Regulators/2(Vq_ref), [Vref]
  [IdIq_ref] -> Selector2/1, Selector/1
  [ModIndex] -> Bus Creator/5  "Mod Index"
  Selector3/1 -> Bus Creator/4  "Iq"
  Constant/1 -> Vref Generation/3(Vdc_meas)
  Bus Creator/1 -> meas/1
  Selector6/1 -> Bus Creator/12  "Vd"
  Selector7/1 -> Bus Creator/13  "Vq"
  [VdVq] -> Selector7/1, Selector6/1
  [Vref] -> Bus Creator/14  "Vref"
  [VdVq] -> Selector10/1, Selector11/1
  Constant1/1 -> Voltage Regulators/5(Vd_ref)
  Selector11/1 -> Voltage Regulators/1(Vq)  "Vq"
  Selector10/1 -> Voltage Regulators/4(Vd)  "Vd"
  Measurements/1(VdVq_meas) -> [VdVq]
  Measurements/2(IdIq_meas) -> [IdIq]
  [IdIq] -> Current Regulator/2(IdIq_meas)
  [VdVq] -> Current Regulator/1(VdVq_meas)
  Droop_On/1 -> Droop Control/5(Enable)
  [Qmeas] -> Unit Delay5/1
  [Pmeas] -> Unit Delay4/1
  Droop Control/3(Fout) -> [Freq]
  Droop Control/1(Vout) -> [Vout]
  Fref/1 -> Droop Control/1(Fref)
  Vref/1 -> Droop Control/2(Vref)
  Droop Control/2(theta_out) -> [wt]
  [wt] -> Vref Generation/1(wt)
  [wt] -> Measurements/4(wt)
  Measurements/3(P_meas) -> [Pmeas]
  Unit Delay/1 -> Vpwm/1
  Unit Delay4/1 -> Droop Control/3(Pmeas)
  Unit Delay5/1 -> Droop Control/4(Qmeas)
  [Freq] -> Measurements/3(Freq)
  Current Regulator/1(VdVq_conv) -> [VdVq_conv]
  [VdVq_conv] -> Vref Generation/2(VdVq_conv)
  Voltage Regulators/1(IdIq_ref) -> [IdIq_ref]

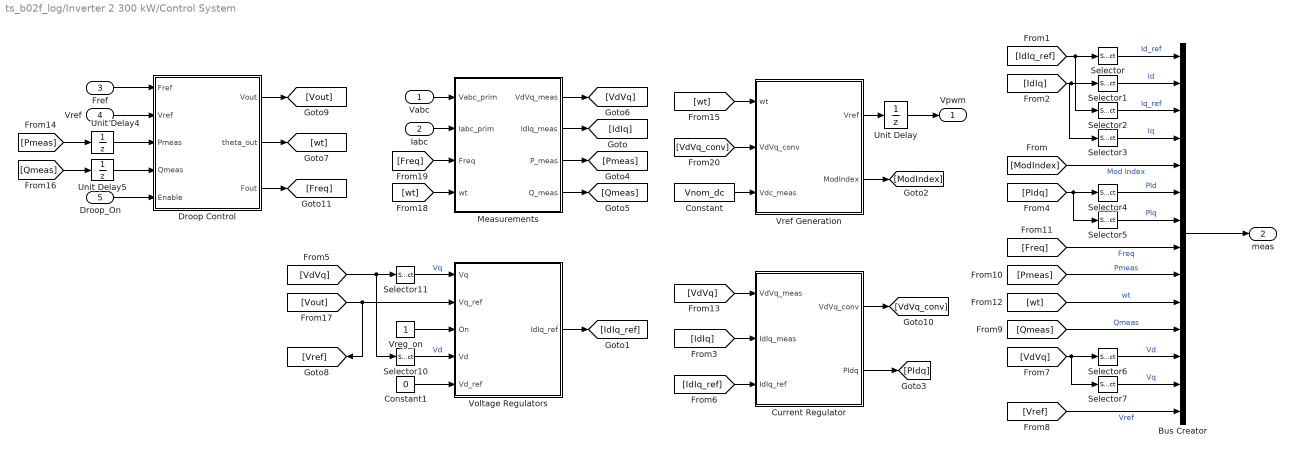
== system ts_b02f_log/Inverter 2 300 kW/Control System ==
  Vabc : Inport  PortDimensions=3
  Iabc : Inport  Port=2  PortDimensions=3
  Fref : Inport  Port=3  PortDimensions=1
  Vref : Inport  Port=4  PortDimensions=1
  Droop_On : Inport  Port=5
  Bus Creator : BusCreator  Inputs=14
  Constant : Constant  Value=Vnom_dc  SampleTime=Ts
  Constant1 : Constant  Value=0  SampleTime=Ts
  Current Regulator : Subsystem
  Droop Control : Subsystem
  Measurements : Subsystem
  Selector{,1,4,6,10} (5 alike) : Selector  InputPortWidth=2  IndexOptions=Index vector (dialog)  Indices=1  OutputSizes=1
  Selector{2..3,5,7,11} (5 alike) : Selector  InputPortWidth=2  IndexOptions=Index vector (dialog)  Indices=2  OutputSizes=1
  Unit Delay : UnitDelay  SampleTime=-1  HasFrameUpgradeWarning=on
  Unit Delay4 : UnitDelay  SampleTime=-1  HasFrameUpgradeWarning=on
  Unit Delay5 : UnitDelay  SampleTime=-1  HasFrameUpgradeWarning=on
  Voltage Regulators : Subsystem
  Vref Generation : Subsystem
  Vreg_on : Constant
  Vpwm : Outport  VectorParamsAs1DForOutWhenUnconnected=off
  meas : Outport  Port=2  VectorParamsAs1DForOutWhenUnconnected=off
  wires:
  Selector1/1 -> Bus Creator/2  "Id"
  Selector5/1 -> Bus Creator/7  "PIq"
  Selector4/1 -> Bus Creator/6  "PId"
  Vref Generation/1(Vref) -> Unit Delay/1
  Iabc/1 -> Measurements/2(Iabc_prim)
  Vref Generation/2(ModIndex) -> [ModIndex]
  Vreg_on/1 -> Voltage Regulators/3(On)
  [IdIq] -> Selector1/1, Selector3/1
  [Qmeas] -> Bus Creator/11  "Qmeas"
  Selector/1 -> Bus Creator/1  "Id_ref"
  [Freq] -> Bus Creator/8  "Freq"
  [wt] -> Bus Creator/10  "wt"
  Selector2/1 -> Bus Creator/3  "Iq_ref"
  Measurements/4(Q_meas) -> [Qmeas]
  [IdIq_ref] -> Current Regulator/3(IdIq_ref)
  [PIdq] -> Selector5/1, Selector4/1
  [Pmeas] -> Bus Creator/9  "Pmeas"
  Vabc/1 -> Measurements/1(Vabc_prim)
  Current Regulator/2(PIdq) -> [PIdq]
  [Vout] -> Voltage Regulators/2(Vq_ref), [Vref]
  [IdIq_ref] -> Selector2/1, Selector/1
  [ModIndex] -> Bus Creator/5  "Mod Index"
  Selector3/1 -> Bus Creator/4  "Iq"
  Constant/1 -> Vref Generation/3(Vdc_meas)
  Bus Creator/1 -> meas/1
  Selector6/1 -> Bus Creator/12  "Vd"
  Selector7/1 -> Bus Creator/13  "Vq"
  [VdVq] -> Selector7/1, Selector6/1
  [Vref] -> Bus Creator/14  "Vref"
  [VdVq] -> Selector10/1, Selector11/1
  Constant1/1 -> Voltage Regulators/5(Vd_ref)
  Selector11/1 -> Voltage Regulators/1(Vq)  "Vq"
  Selector10/1 -> Voltage Regulators/4(Vd)  "Vd"
  Measurements/1(VdVq_meas) -> [VdVq]
  Measurements/2(IdIq_meas) -> [IdIq]
  [IdIq] -> Current Regulator/2(IdIq_meas)
  [VdVq] -> Current Regulator/1(VdVq_meas)
  Droop_On/1 -> Droop Control/5(Enable)
  [Qmeas] -> Unit Delay5/1
  [Pmeas] -> Unit Delay4/1
  Droop Control/3(Fout) -> [Freq]
  Droop Control/1(Vout) -> [Vout]
  Fref/1 -> Droop Control/1(Fref)
  Vref/1 -> Droop Control/2(Vref)
  Droop Control/2(theta_out) -> [wt]
  [wt] -> Vref Generation/1(wt)
  [wt] -> Measurements/4(wt)
  Measurements/3(P_meas) -> [Pmeas]
  Unit Delay/1 -> Vpwm/1
  Unit Delay4/1 -> Droop Control/3(Pmeas)
  Unit Delay5/1 -> Droop Control/4(Qmeas)
  [Freq] -> Measurements/3(Freq)
  Current Regulator/1(VdVq_conv) -> [VdVq_conv]
  [VdVq_conv] -> Vref Generation/2(VdVq_conv)
  Voltage Regulators/1(IdIq_ref) -> [IdIq_ref]

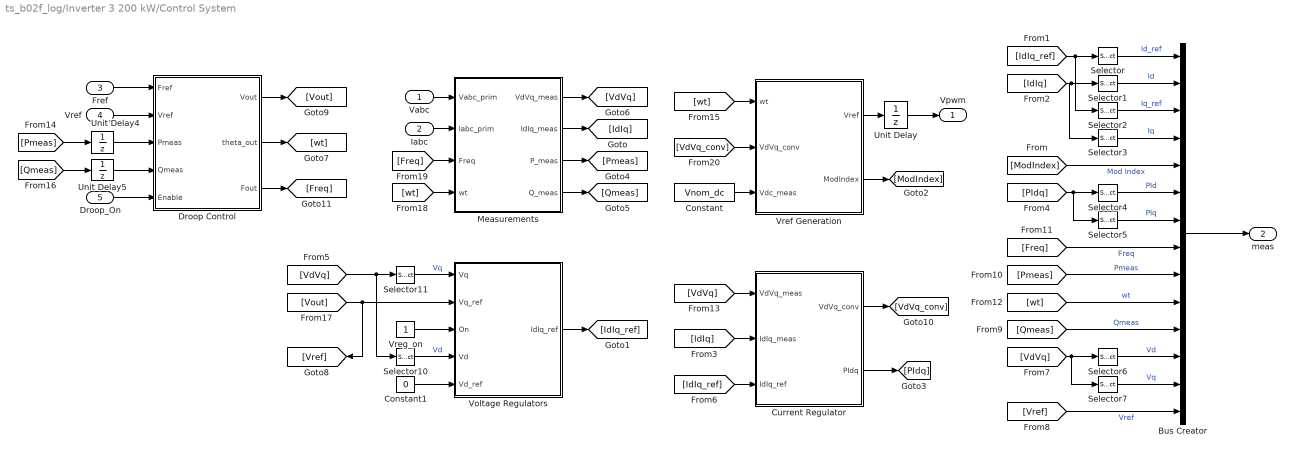
== system ts_b02f_log/Inverter 3 200 kW/Control System ==
  Vabc : Inport  PortDimensions=3
  Iabc : Inport  Port=2  PortDimensions=3
  Fref : Inport  Port=3  PortDimensions=1
  Vref : Inport  Port=4  PortDimensions=1
  Droop_On : Inport  Port=5
  Bus Creator : BusCreator  Inputs=14
  Constant : Constant  Value=Vnom_dc  SampleTime=Ts
  Constant1 : Constant  Value=0  SampleTime=Ts
  Current Regulator : Subsystem
  Droop Control : Subsystem
  Measurements : Subsystem
  Selector{,1,4,6,10} (5 alike) : Selector  InputPortWidth=2  IndexOptions=Index vector (dialog)  Indices=1  OutputSizes=1
  Selector{2..3,5,7,11} (5 alike) : Selector  InputPortWidth=2  IndexOptions=Index vector (dialog)  Indices=2  OutputSizes=1
  Unit Delay : UnitDelay  SampleTime=-1  HasFrameUpgradeWarning=on
  Unit Delay4 : UnitDelay  SampleTime=-1  HasFrameUpgradeWarning=on
  Unit Delay5 : UnitDelay  SampleTime=-1  HasFrameUpgradeWarning=on
  Voltage Regulators : Subsystem
  Vref Generation : Subsystem
  Vreg_on : Constant
  Vpwm : Outport  VectorParamsAs1DForOutWhenUnconnected=off
  meas : Outport  Port=2  VectorParamsAs1DForOutWhenUnconnected=off
  wires:
  Selector1/1 -> Bus Creator/2  "Id"
  Selector5/1 -> Bus Creator/7  "PIq"
  Selector4/1 -> Bus Creator/6  "PId"
  Vref Generation/1(Vref) -> Unit Delay/1
  Iabc/1 -> Measurements/2(Iabc_prim)
  Vref Generation/2(ModIndex) -> [ModIndex]
  Vreg_on/1 -> Voltage Regulators/3(On)
  [IdIq] -> Selector1/1, Selector3/1
  [Qmeas] -> Bus Creator/11  "Qmeas"
  Selector/1 -> Bus Creator/1  "Id_ref"
  [Freq] -> Bus Creator/8  "Freq"
  [wt] -> Bus Creator/10  "wt"
  Selector2/1 -> Bus Creator/3  "Iq_ref"
  Measurements/4(Q_meas) -> [Qmeas]
  [IdIq_ref] -> Current Regulator/3(IdIq_ref)
  [PIdq] -> Selector5/1, Selector4/1
  [Pmeas] -> Bus Creator/9  "Pmeas"
  Vabc/1 -> Measurements/1(Vabc_prim)
  Current Regulator/2(PIdq) -> [PIdq]
  [Vout] -> Voltage Regulators/2(Vq_ref), [Vref]
  [IdIq_ref] -> Selector2/1, Selector/1
  [ModIndex] -> Bus Creator/5  "Mod Index"
  Selector3/1 -> Bus Creator/4  "Iq"
  Constant/1 -> Vref Generation/3(Vdc_meas)
  Bus Creator/1 -> meas/1
  Selector6/1 -> Bus Creator/12  "Vd"
  Selector7/1 -> Bus Creator/13  "Vq"
  [VdVq] -> Selector7/1, Selector6/1
  [Vref] -> Bus Creator/14  "Vref"
  [VdVq] -> Selector10/1, Selector11/1
  Constant1/1 -> Voltage Regulators/5(Vd_ref)
  Selector11/1 -> Voltage Regulators/1(Vq)  "Vq"
  Selector10/1 -> Voltage Regulators/4(Vd)  "Vd"
  Measurements/1(VdVq_meas) -> [VdVq]
  Measurements/2(IdIq_meas) -> [IdIq]
  [IdIq] -> Current Regulator/2(IdIq_meas)
  [VdVq] -> Current Regulator/1(VdVq_meas)
  Droop_On/1 -> Droop Control/5(Enable)
  [Qmeas] -> Unit Delay5/1
  [Pmeas] -> Unit Delay4/1
  Droop Control/3(Fout) -> [Freq]
  Droop Control/1(Vout) -> [Vout]
  Fref/1 -> Droop Control/1(Fref)
  Vref/1 -> Droop Control/2(Vref)
  Droop Control/2(theta_out) -> [wt]
  [wt] -> Vref Generation/1(wt)
  [wt] -> Measurements/4(wt)
  Measurements/3(P_meas) -> [Pmeas]
  Unit Delay/1 -> Vpwm/1
  Unit Delay4/1 -> Droop Control/3(Pmeas)
  Unit Delay5/1 -> Droop Control/4(Qmeas)
  [Freq] -> Measurements/3(Freq)
  Current Regulator/1(VdVq_conv) -> [VdVq_conv]
  [VdVq_conv] -> Vref Generation/2(VdVq_conv)
  Voltage Regulators/1(IdIq_ref) -> [IdIq_ref]

== system ts_b02f_log/Microgrid Supervisory Control/PI regulator with anti-windup q ==
  note: Anti-windup mechanism: Method of conditionnal integration
      |
      | The integration is suspended if saturation occurs and the
      | control error is of the same sign as the control signal.
      |
      | [1] L.Rundqwist, "Anti-Reset Windup for PID Controllers," Ph.D. Thesis TRFT-1033,
      | Departement of Automatic Control, Lund Institute of Technology, Lund, Sweeden, 1991.
  Error : Inport  SampleTime=Ts
  Reset : Inport  Port=2  SampleTime=Ts
  Compare To Zero : simulink/Logic and Bit Operations/Compare To Zero  relop=>  OutDataTypeStr=uint8  ZeroCross=off
  Compare To Zero1 : simulink/Logic and Bit Operations/Compare To Zero  relop=<  OutDataTypeStr=uint8  ZeroCross=off
  Constant : Constant  Value=0
  Constant1 : Constant  Value=UpperLimit
  Constant3 : Constant  Value=LowerLimit
  Discrete-Time Integrator : DiscreteIntegrator  IntegratorMethod=Integration: Trapezoidal  ExternalReset=level  InitialCondition=Init  SampleTime=Ts  LimitOutput=on  UpperSaturationLimit=UpperLimit  LowerSaturationLimit=LowerLimit  ShowStatePort=on  ICPrevOutput=DiscIntNeverNeededParam  ICPrevScaledInput=DiscIntNeverNeededParam
  Kp4 : Gain  Gain=Kp  SaturateOnIntegerOverflow=on  SampleTime=Ts  OutDataTypeStr=Inherit: Same as input  ParamDataTypeStr=Inherit: Same as input
  Kp5 : Gain  Gain=Ki  SaturateOnIntegerOverflow=on  SampleTime=Ts  OutDataTypeStr=Inherit: Same as input  ParamDataTypeStr=Inherit: Same as input
  Logical Operator : Logic  AllPortsSameDT=off  OutDataTypeStr=boolean
  Logical Operator1 : Logic  AllPortsSameDT=off  OutDataTypeStr=boolean
  Logical Operator2 : Logic  Operator=OR  AllPortsSameDT=off  OutDataTypeStr=boolean
  Relational Operator : RelationalOperator  OutDataTypeStr=boolean  InputSameDT=off
  Relational Operator1 : RelationalOperator  Operator=<=  OutDataTypeStr=boolean  InputSameDT=off
  Saturation2 : Saturate  UpperLimit=UpperLimit  LowerLimit=LowerLimit  SampleTime=Ts
  Sum1 : Sum  InputSameDT=on  SaturateOnIntegerOverflow=on  SampleTime=Ts  OutDataTypeStr=Inherit: Same as first input
  Sum6 : Sum  InputSameDT=on  SaturateOnIntegerOverflow=on  SampleTime=Ts  OutDataTypeStr=Inherit: Same as first input
  Switch : Switch  Criteria=u2 > Threshold  SaturateOnIntegerOverflow=off  InputSameDT=off
  Zero-Order Hold : ZeroOrderHold  SampleTime=Ts
  Out : Outport  SampleTime=Ts  InitialOutput=0  VectorParamsAs1DForOutWhenUnconnected=off
  wires:
  Reset/1 -> Discrete-Time Integrator/2
  Constant/1 -> Switch/1
  Zero-Order Hold/1 -> Sum1/2, Sum6/1
  Discrete-Time Integrator/State -> Sum1/1
  Sum1/1 -> Relational Operator1/1, Relational Operator/1
  Logical Operator2/1 -> Switch/2
  Relational Operator/1 -> Logical Operator/1  "UpperLimit_is_Reached"
  Relational Operator1/1 -> Logical Operator1/1  "LowerLimit_Is_Reached"
  Constant1/1 -> Relational Operator/2
  Constant3/1 -> Relational Operator1/2
  Compare To Zero/1 -> Logical Operator/2  "Error_is_positive"
  Logical Operator/1 -> Logical Operator2/1
  Logical Operator1/1 -> Logical Operator2/2
  Compare To Zero1/1 -> Logical Operator1/2  "Error_is_negative"
  Error/1 -> Compare To Zero1/1, Compare To Zero/1, Kp4/1, Kp5/1
  Sum6/1 -> Saturation2/1
  Kp4/1 -> Zero-Order Hold/1
  Discrete-Time Integrator/1 -> Sum6/2
  Saturation2/1 -> Out/1
  Switch/1 -> Discrete-Time Integrator/1
  Kp5/1 -> Switch/3
